simulink library "Battery_Cell_Det_old"  (R2024b)
settings: Solver=ode45  StartTime=0.0  StopTime=10.0  RelTol=1e-3  EnableMultiTasking=on
undefined symbols (not defined in the file or in its folder): HEV_Param, Kt_Temps
libraries: fl_lib x18, LeadAcidBattery_lib x12, nesl_utility x3
Description:
  | Copyright 2014-2024 The MathWorks, Inc.
settings Model: Creator=smiller  LastModifiedBy=smiller
settings SolverCC: AlgebraicLoopSolver=TrustRegion
settings DataIOCC: LimitDataPoints=on  SaveFormat=Array  SignalLoggingSaveFormat=ModelDataLogs  ReturnWorkspaceOutputs=off
settings OptimizationCC: ReuseModelBlockBuffer=off  ExpressionDepthLimit=2147483647  LifeSpan=inf
settings DebuggingCC: UnderspecifiedInitializationDetection=Classic  MergeDetectMultiDrivingBlocksExec=none  SolverPrmCheckMsg=warning  FcnCallInpInsideContextMsg=warning  UnconnectedInputMsg=warning  UnconnectedOutputMsg=warning  UnconnectedLineMsg=warning  AllowSymbolicDim=off  StateNameClashWarn=warning  PregeneratedLibrarySubsystemCodeDiagnostic=none  SFUnexpectedBacktrackingDiag=warning  SFNoUnconditionalDefaultTransitionDiag=warning  SFExecutionAtInitializationDiag=none  ArithmeticOperatorsInVariantConditions=warning
settings HardwareCC: ProdBitPerPointer=32  ProdBitPerSizeT=32  ProdBitPerPtrDiffT=32  ProdLargestAtomicFloat=None  ProdIntDivRoundTo=Undefined  ProdEndianess=Unspecified  ProdWordSize=32  ProdHWDeviceType=32-bit Generic
settings ModelReferenceCC: EnableRefExpFcnMdlSchedulingChecks=on  PropagateSignalLabelsOutOfModel=off
settings SFSimCC: SimUseLocalCustomCode=off  CustomCodeUndefinedFunction=UseInterfaceOnly
settings RTWCC: RTWUseLocalCustomCode=off  GPUComputeCapability=3.5  DLArmComputeVersion=19.05
settings CodeAppCC: StateflowObjectComments=on
settings GRTTargetCC: TargetLangStandard=C89/C90 (ANSI)  CombineOutputUpdateFcns=off  GRTInterface=on
settings ConfigComp: CovMetricSettings=dw  CovSaveCumulativeToWorkspaceVar=on  CovSaveSingleToWorkspaceVar=on  CovExternalEMLEnable=off  CovSFcnEnable=off

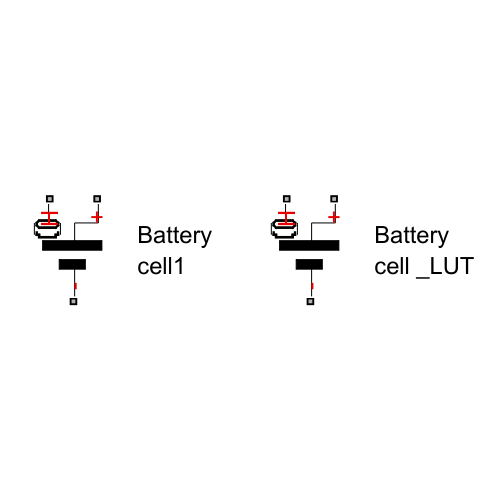
[thumbnail: Simulink's stored preview of the top-level diagram]
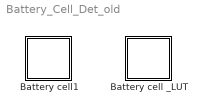
== system Battery_Cell_Det_old ==
  Battery cell _LUT : Subsystem
      mask Display:
      | % Battery icon
      | plot([1.5 0.4],[0 0])
      | plot(-[0.2 0.9 0.9 1.5],[0 0 -0.8 -0.8])
      | patch(([1 1 -1 -1]*0.15-0.5)*-1,[-1 1 1 -1]*0.4,[0;0;0]);
      | patch(([1 1 -1 -1]*0.15+0.1)*-1,[-1 1 1 -1]*0.9,[0;0;0]);
      | 
      | % Thermal port
      | plot([-0.5,-0.9],[1.2,1.2])
      | plot([-0.5,-0.9],[0.4,0.4])
      | plot([-0.9,-1.5],[0.8,0.8])
      | plot(-0.15*sin(0:2*pi/50:2*pi)-0.85,-0.35*cos(0:2*pi/50:2*pi)+0.8)
      | plot(0.15*sin(0:2*pi/50:pi)-0.55,-0.35*cos(0:2*pi/50:pi)+0.8)
      | 
      | % Plot points to set plot range
      | color('white');plot(1.5,1.5);plot(-1.5,-1.5)
      | 
      | color('red')
      | port_label('LConn',1,'H')
      | port_label('LConn',2,'+')
      | port_label('RConn',1,'-')
  Battery cell1 : Subsystem
      mask Display:
      | % Battery icon
      | plot([1.5 0.4],[0 0])
      | plot(-[0.2 0.9 0.9 1.5],[0 0 -0.8 -0.8])
      | patch(([1 1 -1 -1]*0.15-0.5)*-1,[-1 1 1 -1]*0.4,[0;0;0]);
      | patch(([1 1 -1 -1]*0.15+0.1)*-1,[-1 1 1 -1]*0.9,[0;0;0]);
      | 
      | % Thermal port
      | plot([-0.5,-0.9],[1.2,1.2])
      | plot([-0.5,-0.9],[0.4,0.4])
      | plot([-0.9,-1.5],[0.8,0.8])
      | plot(-0.15*sin(0:2*pi/50:2*pi)-0.85,-0.35*cos(0:2*pi/50:2*pi)+0.8)
      | plot(0.15*sin(0:2*pi/50:pi)-0.55,-0.35*cos(0:2*pi/50:pi)+0.8)
      | 
      | % Plot points to set plot range
      | color('white');plot(1.5,1.5);plot(-1.5,-1.5)
      | 
      | color('red')
      | port_label('LConn',1,'H')
      | port_label('LConn',2,'+')
      | port_label('RConn',1,'-')

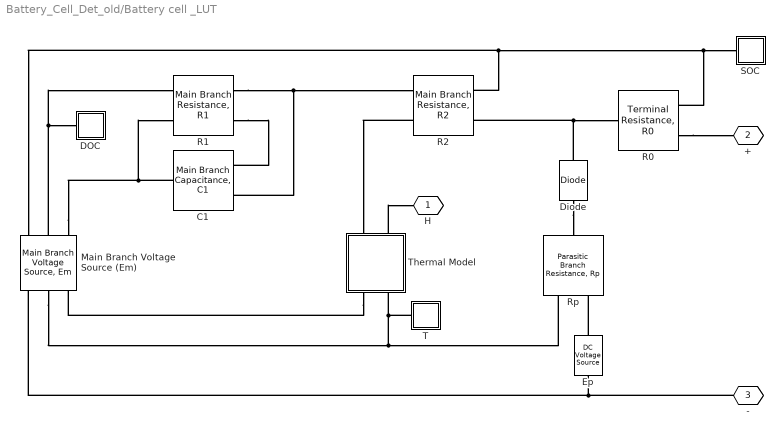
== system Battery_Cell_Det_old/Battery cell _LUT ==
  " DOC " : Subsystem
  " SOC " : Subsystem
  C1 : LeadAcidBattery_lib/Main Branch Capacitance, C1  Tau1=HEV_Param.Battery_Cell.Tau1 s  Cmin=1e-5 F
      settings: InternalSimscapePortConfiguration="{\"Bottom\":[],\"Left\":[{\"id\":\"R1\",\"label\":\"R1\",\"type\":\"input\"},{\"id\":\"p\",\"label\":\"+\",\"type\":\"foundation.electrical.electrical\"}],\"Right\":[{\"id\":\"n\",\"label\":\"-\",\"type\":\"foundation.electrical.electrical\"}],\"Top\":[]}"
  Diode : fl_lib/Electrical/Electrical Elements/Diode  Vf=0.6 V  Ron=0.3 Ohm  Goff=1e-08 1/Ohm  i_specify=off  i_priority=High  i=0 A  i_nominal_specify=off  i_nominal_value=1  i_nominal_unit=A  v_specify=off  v_priority=High  v=0 V  v_nominal_specify=off  v_nominal_value=1  v_nominal_unit=V
  Ep : fl_lib/Electrical/Electrical Sources/DC Voltage Source  v0=HEV_Param.Battery_Cell.Ep V
  Main Branch Voltage Source (Em) : LeadAcidBattery_lib/Main Branch Voltage Source, Em  Em0=HEV_Param.Battery_Cell.Emo V  Ke=HEV_Param.Battery_Cell.Ke V/K  Kc=HEV_Param.Battery_Cell.Kc  C0=HEV_Param.Battery_Cell.Costar s*A  Istar=HEV_Param.Battery_Cell.Istar A  delta=HEV_Param.Battery_Cell.delta  Tau1=HEV_Param.Battery_Cell.Tau1 s  Qinit=HEV_Param.Battery_Cell.Qe_init s*A
      settings: InternalSimscapePortConfiguration="{\"Bottom\":[],\"Left\":[{\"id\":\"SOC\",\"label\":\"SOC\",\"type\":\"output\"},{\"id\":\"DOC\",\"label\":\"DOC\",\"type\":\"output\"},{\"id\":\"p\",\"label\":\"+\",\"type\":\"foundation.electrical.electrical\"}],\"Right\":[{\"id\":\"n\",\"label\":\"-\",\"type\":\"foundation.electrical.electrical\"},{\"id\":\"T\",\"label\":\"T\",\"type\":\"input\"},{\"id\":\"Kt\",\"label\":\"Kt\",\"type\":\"input\"}],\"Top\":[]}"
  R0 : LeadAcidBattery_lib/Terminal Resistance, R0  R00=HEV_Param.Battery_Cell.Roo Ohm  A0=HEV_Param.Battery_Cell.Ao
      settings: InternalSimscapePortConfiguration="{\"Bottom\":[],\"Left\":[{\"id\":\"SOC\",\"label\":\"SOC\",\"type\":\"input\"},{\"id\":\"p\",\"label\":\"+\",\"type\":\"foundation.electrical.electrical\"}],\"Right\":[{\"id\":\"n\",\"label\":\"-\",\"type\":\"foundation.electrical.electrical\"}],\"Top\":[]}"
  R1 : LeadAcidBattery_lib/Main Branch Resistance, R1  R10=HEV_Param.Battery_Cell.R10 Ohm  DOC_min=1e-006
      settings: InternalSimscapePortConfiguration="{\"Bottom\":[],\"Left\":[{\"id\":\"p\",\"label\":\"+\",\"type\":\"foundation.electrical.electrical\"},{\"id\":\"R1\",\"label\":\"R1\",\"type\":\"output\"}],\"Right\":[{\"id\":\"DOC\",\"label\":\"DOC\",\"type\":\"input\"},{\"id\":\"n\",\"label\":\"-\",\"type\":\"foundation.electrical.electrical\"}],\"Top\":[]}"
  R2 : LeadAcidBattery_lib/Main Branch Resistance, R2  R20=HEV_Param.Battery_Cell.R20 Ohm  A21=HEV_Param.Battery_Cell.A21  A22=HEV_Param.Battery_Cell.A22  Istar=HEV_Param.Battery_Cell.Istar A
      settings: InternalSimscapePortConfiguration="{\"Bottom\":[],\"Left\":[{\"id\":\"SOC\",\"label\":\"SOC\",\"type\":\"input\"},{\"id\":\"p\",\"label\":\"+\",\"type\":\"foundation.electrical.electrical\"}],\"Right\":[{\"id\":\"n\",\"label\":\"-\",\"type\":\"foundation.electrical.electrical\"},{\"id\":\"pow\",\"label\":\"POW\",\"type\":\"output\"}],\"Top\":[]}"
  Rp : LeadAcidBattery_lib/Parasitic Branch Resistance, Rp  Gp0=HEV_Param.Battery_Cell.Gpo 1/Ohm  Vp0=HEV_Param.Battery_Cell.Vpo V  Ap=HEV_Param.Battery_Cell.Ap  Tf=HEV_Param.Battery_Cell.theta_f degC
      settings: InternalSimscapePortConfiguration="{\"Bottom\":[],\"Left\":[{\"id\":\"p\",\"label\":\"+\",\"type\":\"foundation.electrical.electrical\"}],\"Right\":[{\"id\":\"theta\",\"label\":\"T\",\"type\":\"input\"},{\"id\":\"n\",\"label\":\"-\",\"type\":\"foundation.electrical.electrical\"}],\"Top\":[]}"
  T : Subsystem
  Thermal Model : Subsystem
  H : PMIOPort  Tag=PMCPort  Side=Left
  + : PMIOPort  Tag=PMCPort  Port=2  Side=Left
  - : PMIOPort  Tag=PMCPort  Port=3  Side=Right
  connections:
  Diode/LConn1 -- R0/RConn1 -- R2/LConn2
  R2/RConn2 -- Thermal Model/LConn1
  -/RConn1 -- Ep/RConn1 -- Main Branch Voltage Source (Em)/RConn1
  Thermal Model/RConn1 -- Main Branch Voltage Source (Em)/RConn3
  Diode/RConn1 -- Rp/LConn1
  Ep/LConn1 -- Rp/RConn2
  Thermal Model/LConn2 -- H/RConn1
  R2/LConn1 -- Main Branch Voltage Source (Em)/LConn1 -- R0/LConn1 -- " SOC "/LConn1
  R1/LConn2 -- C1/LConn1
  R1/LConn1 -- C1/LConn2 -- R2/RConn1
  Main Branch Voltage Source (Em)/LConn3 -- C1/RConn1 -- R1/RConn2
  Main Branch Voltage Source (Em)/LConn2 -- R1/RConn1 -- " DOC "/LConn1
  R0/LConn2 -- +/RConn1
  Main Branch Voltage Source (Em)/RConn2 -- Rp/RConn1 -- T/LConn1 -- Thermal Model/RConn2

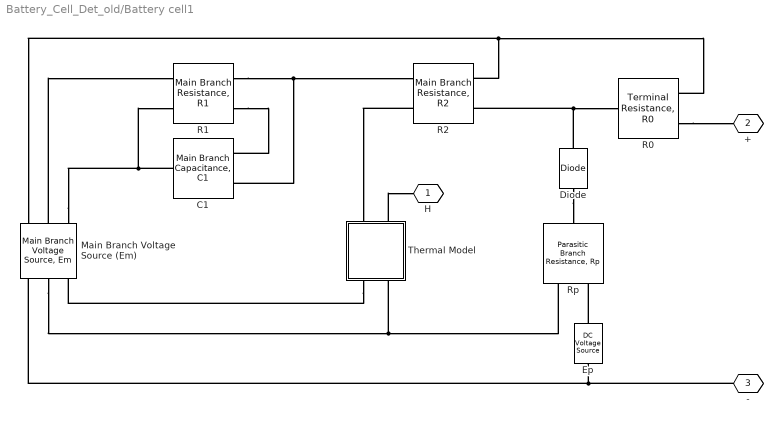
== system Battery_Cell_Det_old/Battery cell1 ==
  C1 : LeadAcidBattery_lib/Main Branch Capacitance, C1  Tau1=HEV_Param.Battery_Cell.Tau1 s  Cmin=1e-5 F
      settings: InternalSimscapePortConfiguration="{\"Bottom\":[],\"Left\":[{\"id\":\"R1\",\"label\":\"R1\",\"type\":\"input\"},{\"id\":\"p\",\"label\":\"+\",\"type\":\"foundation.electrical.electrical\"}],\"Right\":[{\"id\":\"n\",\"label\":\"-\",\"type\":\"foundation.electrical.electrical\"}],\"Top\":[]}"
  Diode : fl_lib/Electrical/Electrical Elements/Diode  Vf=0.6 V  Ron=0.3 Ohm  Goff=1e-08 1/Ohm  i_specify=off  i_priority=High  i=0 A  i_nominal_specify=off  i_nominal_value=1  i_nominal_unit=A  v_specify=off  v_priority=High  v=0 V  v_nominal_specify=off  v_nominal_value=1  v_nominal_unit=V
  Ep : fl_lib/Electrical/Electrical Sources/DC Voltage Source  v0=HEV_Param.Battery_Cell.Ep V
  Main Branch Voltage Source (Em) : LeadAcidBattery_lib/Main Branch Voltage Source, Em  Em0=HEV_Param.Battery_Cell.Emo V  Ke=HEV_Param.Battery_Cell.Ke V/K  Kc=HEV_Param.Battery_Cell.Kc  C0=HEV_Param.Battery_Cell.Costar s*A  Istar=HEV_Param.Battery_Cell.Istar A  delta=HEV_Param.Battery_Cell.delta  Tau1=HEV_Param.Battery_Cell.Tau1 s  Qinit=HEV_Param.Battery_Cell.Qe_init s*A
      settings: InternalSimscapePortConfiguration="{\"Bottom\":[],\"Left\":[{\"id\":\"SOC\",\"label\":\"SOC\",\"type\":\"output\"},{\"id\":\"DOC\",\"label\":\"DOC\",\"type\":\"output\"},{\"id\":\"p\",\"label\":\"+\",\"type\":\"foundation.electrical.electrical\"}],\"Right\":[{\"id\":\"n\",\"label\":\"-\",\"type\":\"foundation.electrical.electrical\"},{\"id\":\"T\",\"label\":\"T\",\"type\":\"input\"},{\"id\":\"Kt\",\"label\":\"Kt\",\"type\":\"input\"}],\"Top\":[]}"
  R0 : LeadAcidBattery_lib/Terminal Resistance, R0  R00=HEV_Param.Battery_Cell.Roo Ohm  A0=HEV_Param.Battery_Cell.Ao
      settings: InternalSimscapePortConfiguration="{\"Bottom\":[],\"Left\":[{\"id\":\"SOC\",\"label\":\"SOC\",\"type\":\"input\"},{\"id\":\"p\",\"label\":\"+\",\"type\":\"foundation.electrical.electrical\"}],\"Right\":[{\"id\":\"n\",\"label\":\"-\",\"type\":\"foundation.electrical.electrical\"}],\"Top\":[]}"
  R1 : LeadAcidBattery_lib/Main Branch Resistance, R1  R10=HEV_Param.Battery_Cell.R10 Ohm  DOC_min=1e-006
      settings: InternalSimscapePortConfiguration="{\"Bottom\":[],\"Left\":[{\"id\":\"p\",\"label\":\"+\",\"type\":\"foundation.electrical.electrical\"},{\"id\":\"R1\",\"label\":\"R1\",\"type\":\"output\"}],\"Right\":[{\"id\":\"DOC\",\"label\":\"DOC\",\"type\":\"input\"},{\"id\":\"n\",\"label\":\"-\",\"type\":\"foundation.electrical.electrical\"}],\"Top\":[]}"
  R2 : LeadAcidBattery_lib/Main Branch Resistance, R2  R20=HEV_Param.Battery_Cell.R20 Ohm  A21=HEV_Param.Battery_Cell.A21  A22=HEV_Param.Battery_Cell.A22  Istar=HEV_Param.Battery_Cell.Istar A
      settings: InternalSimscapePortConfiguration="{\"Bottom\":[],\"Left\":[{\"id\":\"SOC\",\"label\":\"SOC\",\"type\":\"input\"},{\"id\":\"p\",\"label\":\"+\",\"type\":\"foundation.electrical.electrical\"}],\"Right\":[{\"id\":\"n\",\"label\":\"-\",\"type\":\"foundation.electrical.electrical\"},{\"id\":\"pow\",\"label\":\"POW\",\"type\":\"output\"}],\"Top\":[]}"
  Rp : LeadAcidBattery_lib/Parasitic Branch Resistance, Rp  Gp0=HEV_Param.Battery_Cell.Gpo 1/Ohm  Vp0=HEV_Param.Battery_Cell.Vpo V  Ap=HEV_Param.Battery_Cell.Ap  Tf=HEV_Param.Battery_Cell.theta_f degC
      settings: InternalSimscapePortConfiguration="{\"Bottom\":[],\"Left\":[{\"id\":\"p\",\"label\":\"+\",\"type\":\"foundation.electrical.electrical\"}],\"Right\":[{\"id\":\"theta\",\"label\":\"T\",\"type\":\"input\"},{\"id\":\"n\",\"label\":\"-\",\"type\":\"foundation.electrical.electrical\"}],\"Top\":[]}"
  Thermal Model : Subsystem
  H : PMIOPort  Tag=PMCPort  Side=Left
  + : PMIOPort  Tag=PMCPort  Port=2  Side=Left
  - : PMIOPort  Tag=PMCPort  Port=3  Side=Right
  connections:
  Diode/LConn1 -- R0/RConn1 -- R2/LConn2
  R2/RConn2 -- Thermal Model/LConn1
  -/RConn1 -- Ep/RConn1 -- Main Branch Voltage Source (Em)/RConn1
  Thermal Model/RConn1 -- Main Branch Voltage Source (Em)/RConn3
  Diode/RConn1 -- Rp/LConn1
  Ep/LConn1 -- Rp/RConn2
  Thermal Model/LConn2 -- H/RConn1
  R2/LConn1 -- Main Branch Voltage Source (Em)/LConn1 -- R0/LConn1
  R1/LConn2 -- C1/LConn1
  R1/LConn1 -- C1/LConn2 -- R2/RConn1
  Main Branch Voltage Source (Em)/LConn3 -- C1/RConn1 -- R1/RConn2
  Main Branch Voltage Source (Em)/LConn2 -- R1/RConn1
  R0/LConn2 -- +/RConn1
  Main Branch Voltage Source (Em)/RConn2 -- Rp/RConn1 -- Thermal Model/RConn2

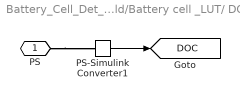
== system Battery_Cell_Det_old/Battery cell _LUT/ DOC  ==
  PS-Simulink Converter1 : nesl_utility/PS-Simulink Converter  PhysicalDomain=network_engine_domain  SubClassName=ps_output  LeftPortType=input  RightPortType=output  PseudoPeriodic=off  Frequencies=[]  VectorFormat=1-D array  Unit=1  AffineConversion=off
  PS : PMIOPort  Side=Left
  tag scope: DOC=global
  wires:
  PS-Simulink Converter1/1 -> [DOC]
  connections:
  PS/RConn1 -- PS-Simulink Converter1/LConn1

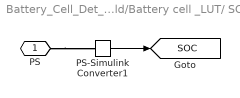
== system Battery_Cell_Det_old/Battery cell _LUT/ SOC  ==
  PS-Simulink Converter1 : nesl_utility/PS-Simulink Converter  PhysicalDomain=network_engine_domain  SubClassName=ps_output  LeftPortType=input  RightPortType=output  PseudoPeriodic=off  Frequencies=[]  VectorFormat=1-D array  Unit=1  AffineConversion=off
  PS : PMIOPort  Side=Left
  tag scope: SOC=global
  wires:
  PS-Simulink Converter1/1 -> [SOC]
  connections:
  PS/RConn1 -- PS-Simulink Converter1/LConn1

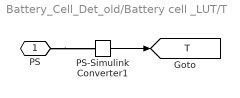
== system Battery_Cell_Det_old/Battery cell _LUT/T ==
  PS-Simulink Converter1 : nesl_utility/PS-Simulink Converter  PhysicalDomain=network_engine_domain  SubClassName=ps_output  LeftPortType=input  RightPortType=output  PseudoPeriodic=off  Frequencies=[]  VectorFormat=1-D array  Unit=degC  AffineConversion=on
  PS : PMIOPort  Side=Left
  tag scope: T=global
  wires:
  PS-Simulink Converter1/1 -> [T]
  connections:
  PS/RConn1 -- PS-Simulink Converter1/LConn1

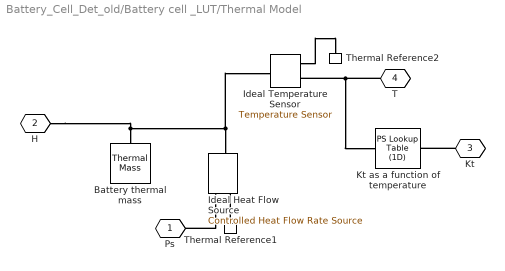
== system Battery_Cell_Det_old/Battery cell _LUT/Thermal Model ==
  Battery thermal mass : fl_lib/Thermal/Thermal Elements/Thermal Mass  mass_type=foundation.enum.constant_variable.constant  mass=1 kg  sp_heat=HEV_Param.Battery_Cell.Ctheta J/kg/K  mass_min=1e-6 kg  num_ports=foundation.enum.numPorts2.one  m_specify=off  m_priority=High  m=1 kg  m_nominal_specify=off  m_nominal_value=1  m_nominal_unit=kg  T_specify=on  T_priority=High  T=HEV_Param.Battery_Cell.theta_init+273 K  T_nominal_specify=off  T_nominal_value=1  T_nominal_unit=K  Q_specify=off  Q_priority=High  Q=0 J/s  Q_nominal_specify=off  Q_nominal_value=1  Q_nominal_unit=J/s
  Ideal Temperature Sensor : fl_lib/Thermal/Thermal Sensors/Temperature Sensor  temperature_measure=foundation.enum.MeasurementReference.difference
  Ideal Heat Flow Source : fl_lib/Thermal/Thermal Sources/Controlled Heat Flow Rate Source
  Kt as a function of temperature : fl_lib/Physical Signals/Lookup Tables/PS Lookup Table (1D)  x=[HEV_Param.Battery_Cell.theta_f,HEV_Param.Battery_Cell. Kt_Temps]+273 K  f=[0 HEV_Param.Battery_Cell.Kt]  interp_method=simscape.enum.interpolation.linear  extrap_method=simscape.enum.extrapolation.linear
  Thermal Reference1 : fl_lib/Thermal/Thermal Elements/Thermal Reference
  Thermal Reference2 : fl_lib/Thermal/Thermal Elements/Thermal Reference
  Ps : PMIOPort  Tag=PMCPort  Side=Left
  H : PMIOPort  Tag=PMCPort  Port=2  Side=Left
  Kt : PMIOPort  Tag=PMCPort  Port=3  Side=Right
  T : PMIOPort  Tag=PMCPort  Port=4  Side=Right
  connections:
  Ideal Heat Flow Source/RConn1 -- Ps/RConn1
  Kt/RConn1 -- Kt as a function of temperature/RConn1
  Battery thermal mass/LConn1 -- Ideal Heat Flow Source/LConn1 -- Ideal Temperature Sensor/LConn1 -- H/RConn1
  Thermal Reference1/LConn1 -- Ideal Heat Flow Source/RConn2
  T/RConn1 -- Kt as a function of temperature/LConn1 -- Ideal Temperature Sensor/RConn2
  Ideal Temperature Sensor/RConn1 -- Thermal Reference2/LConn1

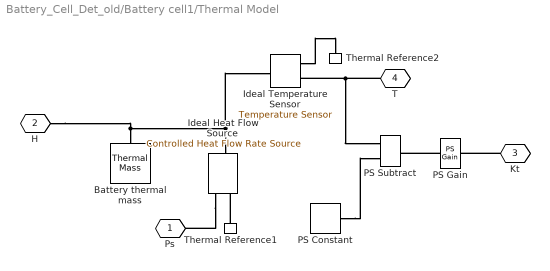
== system Battery_Cell_Det_old/Battery cell1/Thermal Model ==
  Battery thermal mass : fl_lib/Thermal/Thermal Elements/Thermal Mass  mass_type=foundation.enum.constant_variable.constant  mass=1 kg  sp_heat=HEV_Param.Battery_Cell.Ctheta J/kg/K  mass_min=1e-6 kg  num_ports=foundation.enum.numPorts2.one  m_specify=off  m_priority=High  m=1 kg  m_nominal_specify=off  m_nominal_value=1  m_nominal_unit=kg  T_specify=on  T_priority=High  T=HEV_Param.Battery_Cell.theta_init+273 K  T_nominal_specify=off  T_nominal_value=1  T_nominal_unit=K  Q_specify=off  Q_priority=High  Q=0 J/s  Q_nominal_specify=off  Q_nominal_value=1  Q_nominal_unit=J/s
  Ideal Temperature Sensor : fl_lib/Thermal/Thermal Sensors/Temperature Sensor  temperature_measure=foundation.enum.MeasurementReference.difference
  Ideal Heat Flow Source : fl_lib/Thermal/Thermal Sources/Controlled Heat Flow Rate Source
  PS Constant : fl_lib/Physical Signals/Sources/PS Constant  constant=2.89 K
  PS Gain : fl_lib/Physical Signals/Functions/PS Gain  gain=0.0123 1/K
  PS Subtract : fl_lib/Physical Signals/Functions/PS Subtract
  Thermal Reference1 : fl_lib/Thermal/Thermal Elements/Thermal Reference
  Thermal Reference2 : fl_lib/Thermal/Thermal Elements/Thermal Reference
  Ps : PMIOPort  Tag=PMCPort  Side=Left
  H : PMIOPort  Tag=PMCPort  Port=2  Side=Left
  Kt : PMIOPort  Tag=PMCPort  Port=3  Side=Right
  T : PMIOPort  Tag=PMCPort  Port=4  Side=Right
  connections:
  PS Gain/LConn1 -- PS Subtract/RConn1
  PS Constant/RConn1 -- PS Subtract/LConn2
  Ideal Heat Flow Source/RConn1 -- Ps/RConn1
  Kt/RConn1 -- PS Gain/RConn1
  Battery thermal mass/LConn1 -- Ideal Heat Flow Source/LConn1 -- Ideal Temperature Sensor/LConn1 -- H/RConn1
  Thermal Reference1/LConn1 -- Ideal Heat Flow Source/RConn2
  T/RConn1 -- Ideal Temperature Sensor/RConn2 -- PS Subtract/LConn1
  Ideal Temperature Sensor/RConn1 -- Thermal Reference2/LConn1
